simulink model "H06_Tekercs"  (R2026a)
settings: Solver=VariableStepAuto  StopTime=10e-3
settings Model: Creator=Szalay  LastModifiedBy=Szalay

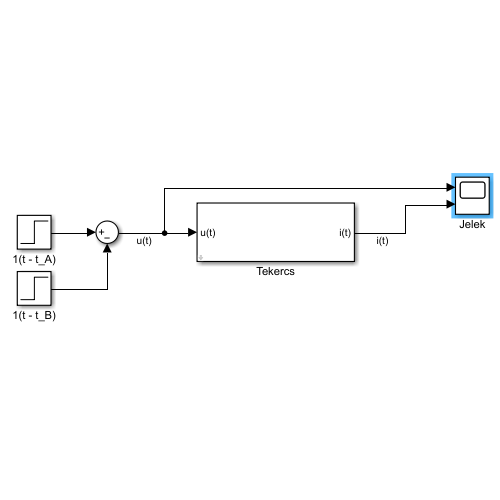
[thumbnail: Simulink's stored preview of the top-level diagram]
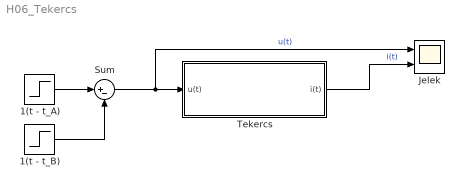
== system H06_Tekercs ==
  1(t - t_A) : Step  Time=2e-3  SampleTime=0
  1(t - t_B) : Step  Time=6e-3  SampleTime=0
  Jelek : Scope  NumInputPorts=2
      settings: ActiveDisplayYMinimum=-0.12499999999999997  ActiveDisplayYMaximum=1.125
  Sum : Sum  Inputs=|+-
  Tekercs : Subsystem  mask(Tekercs){R=1, L=1e-3, i_0=0}
      mask prompts: R "Ellenállás"; L "Öninduktivitás"; i_0 "Kezdeti áramerősség"
      mask help: Soros RL-tag alapú lineáris tekercsmodell.
      mask DialogControl ParameterGroupVar Prompt: Modellparaméterek
      mask DialogControl Container3 Prompt: Kezdeti érték
  wires:
  1(t - t_A)/1 -> Sum/1
  1(t - t_B)/1 -> Sum/2
  Sum/1 -> Jelek/1, Tekercs/1(u(t))  "u(t)"
  Tekercs/1(i(t)) -> Jelek/2  "i(t)"

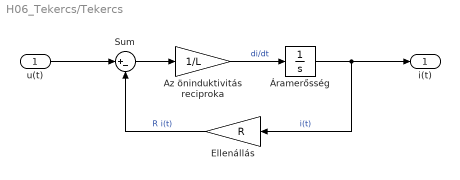
== system H06_Tekercs/Tekercs ==
  u(t) : Inport
  Az öninduktivitás reciproka : Gain  Gain=1/L
  Ellenállás : Gain  Gain=R
  Sum : Sum  Inputs=|+-
  Áramerősség : Integrator  InitialCondition=i_0
  i(t) : Outport
  wires:
  u(t)/1 -> Sum/1
  Sum/1 -> Az öninduktivitás reciproka/1
  Áramerősség/1 -> i(t)/1, Ellenállás/1  "i(t)"
  Ellenállás/1 -> Sum/2  "R i(t)"
  Az öninduktivitás reciproka/1 -> Áramerősség/1  "di/dt"
